simulink model "t_drone"  (R2025b)
settings: Solver=ode23t  StartTime=0.0  StopTime=timespot_spl(end)+2  FixedStep=0.01  MaxStep=1e-2  MinStep=1e-13  RelTol=1e-3  AbsTol=1e-3
InitFcn:
  | model = gcs;
  | 
  | configs = evalin('base', get_param([model '/Configurations'], 'Value'));
  | hold_time = evalin('base', get_param([model '/Hold Time'], 'Value'));
  | transistion_time = evalin('base', get_param([model '/Transistion Time'], 'Value'));
  | 
  | if exist('transforms', 'var') == 1
  |     transforms = transforms;
  | else
  |     transforms = false;
  | end
  | 
  | set_drone_configurations
model workspace (MATLAB code in the model file):
  | load('xy_data_membrane.mat');
undefined symbols (not defined in the file): air_rho, battery, drone_leg, filtD_altitude, filtD_attitude, filtD_motor, filtD_pitch, filtD_position, filtD_roll, filtD_yaw, filtM_altitude, filtM_attitude, filtM_pitch, filtM_position, filtM_roll, filtM_yaw, filtSpd_motor, kd_altitude, kd_attitude, kd_motor, kd_pitch, kd_position, kd_roll, kd_yaw, ki_altitude, ki_attitude, ki_motor, ki_pitch, ki_position, ki_roll, ki_yaw, kp_altitude, kp_attitude, kp_motor, kp_pitch, kp_position, kp_roll, kp_yaw, limit_altitude, limit_attitude, limit_motor, limit_pitch, limit_roll, limit_yaw, mass, pkgDensity, pkgSize, planedepth, pos2attitude, propeller, qc_motor, qd_area, qd_drag, spline_data, spline_yaw, timespot_spl, timespots, waypoints, wind_speed, X ... (+2)
libraries: sm_lib x176, nesl_utility x46, fl_lib x37, slpidlib x9, ee_lib x5, simulink_extras x4, sdl_lib x4, simulink x2, batteryecm_lib x1
(part 4 of 8)

== system t_drone/Quadcopter/Ground ==
  Ground : Subsystem  mask{waypoints=waypoints}
      mask prompts: waypoints "Waypoints [xyz] (m)"
      mask init:
      | plane_x = max(waypoints(1,:))-min(waypoints(1,:))+6;
      | plane_y = max(waypoints(2,:))-min(waypoints(2,:))+6;
      | 
      | offset_x = plane_x/2+min(waypoints(1,:))-3;
      | offset_y = plane_y/2+min(waypoints(2,:))-3;
  Infinite Plane : sm_lib/Curves and Surfaces/Infinite Plane  GraphicType=None  GraphicPlaneWidth=1  GraphicPlaneWidthUnits=m  GraphicPlaneHeight=1  GraphicPlaneHeightUnits=m  GraphicVisPropType=SimpleVisualProperties  GraphicDiffuseColor=[0.5 0.5 0.5]  GraphicOpacity=0  GraphicSpecularColor=[0.5 0.5 0.5 1.0]  GraphicAmbientColor=[0.15 0.15 0.15 1.0]  GraphicEmissiveColor=[0.0 0.0 0.0 1.0]  GraphicShininess=75
  Launch Insignia : sm_lib/Body Elements/Extruded Solid  ExtrusionType=General  PolygonNumSides=3  PolygonOuterRadius=1  PolygonOuterRadiusUnits=m  ExportEntireGeometry=off  ExtrusionCrossSection=[0.15 0.15; -0.15 0.15; -0.15 0.75; -0.6 0.75; -0.6 -0.75; -0.15 -0.75; -0.15 -0.15; 0.15 -0.15; 0.15 -0.75; 0.6 -0.75; 0.6 0.75; 0.15 0.75]*0.5  ExtrusionCrossSectionUnits=m  ExportConvexHullGeometry=off  ExtrusionLength=0.002  ExtrusionLengthUnits=m  InertiaType=CalculateFromGeometry  BasedOnType=Density  Density=1  DensityUnits=kg/m^3  Mass=1  MassUnits=kg  CenterOfMass=[0 0 0]  CenterOfMassUnits=m  MomentsOfInertia=[1 1 1]  MomentsOfInertiaUnits=kg*m^2  ProductsOfInertia=[0 0 0]  ProductsOfInertiaUnits=kg*m^2  GraphicType=FromGeometry  MarkerShape=Sphere  MarkerSize=10  GraphicVisPropType=SimpleVisualProperties  GraphicDiffuseColor=[0.3 0.3 0.3]  GraphicOpacity=1.0  GraphicSpecularColor=[0.5 0.5 0.5 1.0]  GraphicAmbientColor=[0.15 0.15 0.15 1.0]  GraphicEmissiveColor=[0.0 0.0 0.0 1.0]  GraphicShininess=75  DoExposeReferenceFrame=on  SerializedFrames=<Frames/>
  Launch Ring : sm_lib/Body Elements/Revolved Solid  RevolutionCrossSection=[0.5 0.001; 0.5 -0.001; 0.75 -0.001; 0.75 0.001]  RevolutionCrossSectionUnits=m  RevolutionExtent=Full  RevolutionAngle=180  RevolutionAngleUnits=deg  ExportConvexHullGeometry=off  InertiaType=CalculateFromGeometry  BasedOnType=Density  Density=1000  DensityUnits=kg/m^3  Mass=1  MassUnits=kg  CenterOfMass=[0 0 0]  CenterOfMassUnits=m  MomentsOfInertia=[1 1 1]  MomentsOfInertiaUnits=kg*m^2  ProductsOfInertia=[0 0 0]  ProductsOfInertiaUnits=kg*m^2  GraphicType=FromGeometry  MarkerShape=Sphere  MarkerSize=10  GraphicVisPropType=SimpleVisualProperties  GraphicDiffuseColor=[0.3 0.3 0.3]  GraphicOpacity=1.0  GraphicSpecularColor=[0.5 0.5 0.5 1.0]  GraphicAmbientColor=[0.15 0.15 0.15 1.0]  GraphicEmissiveColor=[0.0 0.0 0.0 1.0]  GraphicShininess=75  DoExposeReferenceFrame=on  SerializedFrames=<Frames/>
  Obstacles2 : Subsystem  VariantControl=show_obstacles
  Target Inner Ring : sm_lib/Body Elements/Revolved Solid  RevolutionCrossSection=[0.5 0.001; 0.5 -0.001; 0.75 -0.001; 0.75 0.001]*0.25  RevolutionCrossSectionUnits=m  RevolutionExtent=Full  RevolutionAngle=180  RevolutionAngleUnits=deg  ExportConvexHullGeometry=off  InertiaType=CalculateFromGeometry  BasedOnType=Density  Density=1000  DensityUnits=kg/m^3  Mass=1  MassUnits=kg  CenterOfMass=[0 0 0]  CenterOfMassUnits=m  MomentsOfInertia=[1 1 1]  MomentsOfInertiaUnits=kg*m^2  ProductsOfInertia=[0 0 0]  ProductsOfInertiaUnits=kg*m^2  GraphicType=FromGeometry  MarkerShape=Sphere  MarkerSize=10  GraphicVisPropType=SimpleVisualProperties  GraphicDiffuseColor=[1.0 0.2 0.2]  GraphicOpacity=1.0  GraphicSpecularColor=[0.5 0.5 0.5 1.0]  GraphicAmbientColor=[0.15 0.15 0.15 1.0]  GraphicEmissiveColor=[0.0 0.0 0.0 1.0]  GraphicShininess=75  DoExposeReferenceFrame=on  SerializedFrames=<Frames/>
  Target Middle Ring : sm_lib/Body Elements/Revolved Solid  RevolutionCrossSection=[0.5 0.001; 0.5 -0.001; 0.75 -0.001; 0.75 0.001]*0.5  RevolutionCrossSectionUnits=m  RevolutionExtent=Full  RevolutionAngle=180  RevolutionAngleUnits=deg  ExportConvexHullGeometry=off  InertiaType=CalculateFromGeometry  BasedOnType=Density  Density=1000  DensityUnits=kg/m^3  Mass=1  MassUnits=kg  CenterOfMass=[0 0 0]  CenterOfMassUnits=m  MomentsOfInertia=[1 1 1]  MomentsOfInertiaUnits=kg*m^2  ProductsOfInertia=[0 0 0]  ProductsOfInertiaUnits=kg*m^2  GraphicType=FromGeometry  MarkerShape=Sphere  MarkerSize=10  GraphicVisPropType=SimpleVisualProperties  GraphicDiffuseColor=[1.0 0.8 0.2]  GraphicOpacity=1.0  GraphicSpecularColor=[0.5 0.5 0.5 1.0]  GraphicAmbientColor=[0.15 0.15 0.15 1.0]  GraphicEmissiveColor=[0.0 0.0 0.0 1.0]  GraphicShininess=75  DoExposeReferenceFrame=on  SerializedFrames=<Frames/>
  Target Outer Ring : sm_lib/Body Elements/Revolved Solid  RevolutionCrossSection=[0.5 0.001; 0.5 -0.001; 0.75 -0.001; 0.75 0.001]  RevolutionCrossSectionUnits=m  RevolutionExtent=Full  RevolutionAngle=180  RevolutionAngleUnits=deg  ExportConvexHullGeometry=off  InertiaType=CalculateFromGeometry  BasedOnType=Density  Density=1000  DensityUnits=kg/m^3  Mass=1  MassUnits=kg  CenterOfMass=[0 0 0]  CenterOfMassUnits=m  MomentsOfInertia=[1 1 1]  MomentsOfInertiaUnits=kg*m^2  ProductsOfInertia=[0 0 0]  ProductsOfInertiaUnits=kg*m^2  GraphicType=FromGeometry  MarkerShape=Sphere  MarkerSize=10  GraphicVisPropType=SimpleVisualProperties  GraphicDiffuseColor=[0.2 0.4 1.0]  GraphicOpacity=1.0  GraphicSpecularColor=[0.5 0.5 0.5 1.0]  GraphicAmbientColor=[0.15 0.15 0.15 1.0]  GraphicEmissiveColor=[0.0 0.0 0.0 1.0]  GraphicShininess=75  DoExposeReferenceFrame=on  SerializedFrames=<Frames/>
  Trajectory : Subsystem
  Transform Launch : sm_lib/Frames and Transforms/Rigid Transform  RotationMethod=None  FollAlignAxisA=+X  BaseAlignAxisA=+Y  FollAlignAxisB=+Y  BaseAlignAxisB=+Z  RotationStandardAxis=+Z  RotationAngle=0.0  RotationAngleUnits=deg  RotationArbitraryAxis=[0 0 1]  RotationSequenceAxes=FollowerAxes  RotationSequence=XYX  RotationSequenceAngles=[0 0 0]  RotationSequenceAnglesUnits=deg  RotationMatrix=[1 0 0; 0 1 0; 0 0 1]  Quaternion=[1 0 0 0]  TranslationMethod=Cartesian  TranslationCartesianOffset=[waypoints(1:2,1)' 0 ]  TranslationCartesianOffsetUnits=m  TranslationStandardAxis=+Z  TranslationStandardOffset=0  TranslationStandardOffsetUnits=m  TranslationROffset=0  TranslationROffsetUnits=m  TranslationThetaOffset=0  TranslationThetaOffsetUnits=deg  TranslationZOffset=0  TranslationZOffsetUnits=m
  Transform Target : sm_lib/Frames and Transforms/Rigid Transform  RotationMethod=None  FollAlignAxisA=+X  BaseAlignAxisA=+Y  FollAlignAxisB=+Y  BaseAlignAxisB=+Z  RotationStandardAxis=+Z  RotationAngle=0.0  RotationAngleUnits=deg  RotationArbitraryAxis=[0 0 1]  RotationSequenceAxes=FollowerAxes  RotationSequence=XYX  RotationSequenceAngles=[0 0 0]  RotationSequenceAnglesUnits=deg  RotationMatrix=[1 0 0; 0 1 0; 0 0 1]  Quaternion=[1 0 0 0]  TranslationMethod=Cartesian  TranslationCartesianOffset=[waypoints(1:2,end)' 0 ]  TranslationCartesianOffsetUnits=m  TranslationStandardAxis=+Z  TranslationStandardOffset=0  TranslationStandardOffsetUnits=m  TranslationROffset=0  TranslationROffsetUnits=m  TranslationThetaOffset=0  TranslationThetaOffsetUnits=deg  TranslationZOffset=0  TranslationZOffsetUnits=m
  Variant Connector : VariantPMConnector  VariantControls=__PRM__SERIALIZED__DATA__:show_obstacles == true
  W : PMIOPort  Side=Right
  G : PMIOPort  Port=2  Side=Left
  connections:
  W/RConn1 -- Ground/LConn1 -- Transform Launch/LConn1 -- Transform Target/LConn1 -- Trajectory/RConn1
  Target Middle Ring/RConn1 -- Target Inner Ring/RConn1 -- Transform Target/RConn1 -- Target Outer Ring/RConn1
  Infinite Plane/LConn1 -- Ground/RConn1
  Infinite Plane/RConn1 -- G/RConn1
  Launch Ring/RConn1 -- Variant Connector/RConn1 -- Transform Launch/RConn1 -- Launch Insignia/RConn1
  Variant Connector/LConn1 -- Obstacles2/LConn1

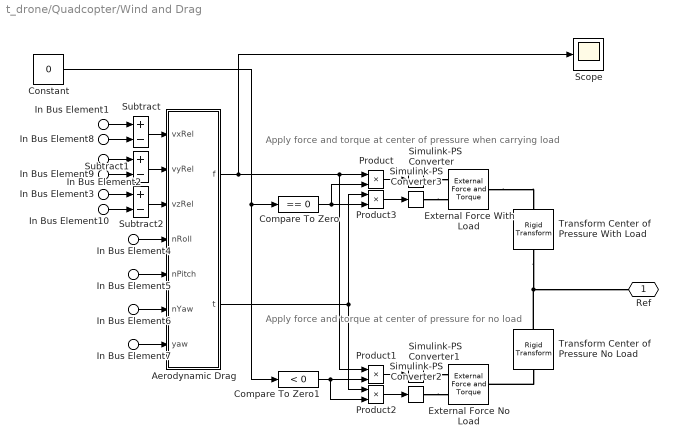
== system t_drone/Quadcopter/Wind and Drag ==
  note: Apply force and torque at center of pressure when carrying load
  note: Apply force and torque at center of pressure for no load
  In Bus Element8 : Inport  PortName=Env  Element=vx
  In Bus Element9 : Inport  PortName=Env  Element=vy
  In Bus Element10 : Inport  PortName=Env  Element=vz
  In Bus Element1 : Inport  Port=2  PortName=Cha  Element=vx
  In Bus Element2 : Inport  Port=2  PortName=Cha  Element=vy
  In Bus Element3 : Inport  Port=2  PortName=Cha  Element=vz
  In Bus Element4 : Inport  Port=2  PortName=Cha  Element=nRoll
  In Bus Element5 : Inport  Port=2  PortName=Cha  Element=nPitch
  In Bus Element6 : Inport  Port=2  PortName=Cha  Element=nYaw
  In Bus Element7 : Inport  Port=2  PortName=Cha  Element=yaw
  Aerodynamic Drag : Subsystem  mask{drag_coeff=qd_drag, area_values=qd_area, rho_air=air_rho}
      mask prompts: drag_coeff "Drag Coefficients"; area_values "Area Values (m^2)"; rho_air "Air Density"
  Compare To Zero : simulink/Logic and Bit Operations/Compare To Zero  relop===  OutDataTypeStr=uint8  ZeroCross=off
  Compare To Zero1 : simulink/Logic and Bit Operations/Compare To Zero  relop=<  OutDataTypeStr=uint8  ZeroCross=off
  Constant : Constant  Value=0
  External Force No Load : sm_lib/Forces and Torques/External Force and Torque  EnableForceX=off  EnableForceY=off  EnableForceZ=off  EnableForce=on  ForceResolutionFrame=World  EnableTorqueX=off  EnableTorqueY=off  EnableTorqueZ=off  EnableTorque=on  TorqueResolutionFrame=AttachedFrame
  External Force With Load : sm_lib/Forces and Torques/External Force and Torque  EnableForceX=off  EnableForceY=off  EnableForceZ=off  EnableForce=on  ForceResolutionFrame=World  EnableTorqueX=off  EnableTorqueY=off  EnableTorqueZ=off  EnableTorque=on  TorqueResolutionFrame=AttachedFrame
  Product{,1..3} (4 alike) : Product
  Scope : Scope
      settings: ActiveDisplayYMinimum=-0.40984  ActiveDisplayYMaximum=3.52459
  Simulink-PS Converter{,1..3} (4 alike) : nesl_utility/Simulink-PS Converter  PhysicalDomain=network_engine_domain  SubClassName=ps_input  LeftPortType=input  RightPortType=output  PseudoPeriodic=off  Frequencies=[]  NoiseDistribution=none  NoiseParameters=[]  Unit=1  AffineConversion=off  FilteringAndDerivatives=provide  SimscapeFilterOrder=1  InputFilterTimeConstant=0.001  UdotUserProvided=0
  Subtract : Sum  Inputs=+-
  Subtract1 : Sum  Inputs=+-
  Subtract2 : Sum  Inputs=+-
  Transform Center of Pressure No Load : sm_lib/Frames and Transforms/Rigid Transform  RotationMethod=None  FollAlignAxisA=+X  BaseAlignAxisA=+Y  FollAlignAxisB=+Y  BaseAlignAxisB=+Z  RotationStandardAxis=+Z  RotationAngle=0.0  RotationAngleUnits=deg  RotationArbitraryAxis=[0 0 1]  RotationSequenceAxes=FollowerAxes  RotationSequence=XYX  RotationSequenceAngles=[0 0 0]  RotationSequenceAnglesUnits=deg  RotationMatrix=[1 0 0; 0 1 0; 0 0 1]  Quaternion=[1 0 0 0]  TranslationMethod=None  TranslationCartesianOffset=[0 0 0]  TranslationCartesianOffsetUnits=m  TranslationStandardAxis=+Z  TranslationStandardOffset=0  TranslationStandardOffsetUnits=m  TranslationROffset=0  TranslationROffsetUnits=m  TranslationThetaOffset=0  TranslationThetaOffsetUnits=deg  TranslationZOffset=0  TranslationZOffsetUnits=m
  Transform Center of Pressure With Load : sm_lib/Frames and Transforms/Rigid Transform  RotationMethod=None  FollAlignAxisA=+X  BaseAlignAxisA=+Y  FollAlignAxisB=+Y  BaseAlignAxisB=+Z  RotationStandardAxis=+Z  RotationAngle=0.0  RotationAngleUnits=deg  RotationArbitraryAxis=[0 0 1]  RotationSequenceAxes=FollowerAxes  RotationSequence=XYX  RotationSequenceAngles=[0 0 0]  RotationSequenceAnglesUnits=deg  RotationMatrix=[1 0 0; 0 1 0; 0 0 1]  Quaternion=[1 0 0 0]  TranslationMethod=StandardAxis  TranslationCartesianOffset=[0 0 0]  TranslationCartesianOffsetUnits=m  TranslationStandardAxis=+Z  TranslationStandardOffset=-pkgSize(3)/2  TranslationStandardOffsetUnits=m  TranslationROffset=0  TranslationROffsetUnits=m  TranslationThetaOffset=0  TranslationThetaOffsetUnits=deg  TranslationZOffset=0  TranslationZOffsetUnits=m
  Ref : PMIOPort  Side=Right
  wires:
  Product/1 -> Simulink-PS Converter/1
  Product1/1 -> Simulink-PS Converter1/1
  Constant/1 -> Compare To Zero1/1, Compare To Zero/1
  Compare To Zero/1 -> Product/2, Product3/2
  Compare To Zero1/1 -> Product2/2, Product1/2
  In Bus Element1/1 -> Subtract/1
  In Bus Element8/1 -> Subtract/2
  In Bus Element7/1 -> Aerodynamic Drag/7(yaw)
  In Bus Element2/1 -> Subtract1/1
  In Bus Element9/1 -> Subtract1/2
  Subtract/1 -> Aerodynamic Drag/1(vxRel)
  Subtract1/1 -> Aerodynamic Drag/2(vyRel)
  In Bus Element3/1 -> Subtract2/1
  In Bus Element10/1 -> Subtract2/2
  Subtract2/1 -> Aerodynamic Drag/3(vzRel)
  In Bus Element4/1 -> Aerodynamic Drag/4(nRoll)
  In Bus Element5/1 -> Aerodynamic Drag/5(nPitch)
  In Bus Element6/1 -> Aerodynamic Drag/6(nYaw)
  Product2/1 -> Simulink-PS Converter2/1
  Product3/1 -> Simulink-PS Converter3/1
  Aerodynamic Drag/1(f) -> Scope/1, Product1/1, Product/1
  Aerodynamic Drag/2(t) -> Product3/1, Product2/1
  connections:
  Transform Center of Pressure With Load/LConn1 -- Transform Center of Pressure No Load/LConn1 -- Ref/RConn1
  Transform Center of Pressure No Load/RConn1 -- External Force No Load/RConn1
  External Force With Load/RConn1 -- Transform Center of Pressure With Load/RConn1
  Simulink-PS Converter/RConn1 -- External Force With Load/LConn1
  Simulink-PS Converter1/RConn1 -- External Force No Load/LConn1
  Simulink-PS Converter2/RConn1 -- External Force No Load/LConn2
  Simulink-PS Converter3/RConn1 -- External Force With Load/LConn2

== system t_drone/Reference/Derivative ==
  des xyz : Inport
  Demux : Demux  Outputs=3
  Derivative : Derivative
  Derivative1 : Derivative
  Derivative2 : Derivative
  Mux1 : Mux  Inputs=3
  des_vel : Outport
  wires:
  Demux/1 -> Derivative/1
  Mux1/1 -> des_vel/1  "des_vel"
  des xyz/1 -> Demux/1
  Demux/2 -> Derivative1/1
  Demux/3 -> Derivative2/1
  Derivative2/1 -> Mux1/3
  Derivative/1 -> Mux1/1
  Derivative1/1 -> Mux1/2

== system t_drone/Reference/Interpolate Spline Points ==
  In1 : Inport
  Constant : Constant  Value=timespot_spl(end)
  Lookup Linear Interpolation1 : Lookup_n-D  NumberOfTableDimensions=1  BreakpointsForDimension1=timespot_spl  Table=spline_yaw  InterpMethod=Akima spline  ExtrapMethod=Clip  InternalRulePriority=Speed  RndMeth=Simplest
  Lookup Linear Interpolation4 : Lookup_n-D  NumberOfTableDimensions=1  BreakpointsForDimension1=timespot_spl  Table=spline_data(:,1)  InterpMethod=Cubic spline  ExtrapMethod=Clip  InternalRulePriority=Speed  RndMeth=Simplest
  Lookup Linear Interpolation5 : Lookup_n-D  NumberOfTableDimensions=1  BreakpointsForDimension1=timespot_spl  Table=spline_data(:,2)  InterpMethod=Cubic spline  ExtrapMethod=Clip  InternalRulePriority=Speed  RndMeth=Simplest
  Lookup Linear Interpolation6 : Lookup_n-D  NumberOfTableDimensions=1  BreakpointsForDimension1=timespot_spl  Table=spline_data(:,3)  InterpMethod=Cubic spline  ExtrapMethod=Clip  InternalRulePriority=Speed  RndMeth=Simplest
  Min : MinMax  Inputs=2
  Mux2 : Mux  Inputs=3
  Yaw : Outport
  des_pos : Outport  Port=2
  wires:
  Mux2/1 -> des_pos/1  "des_pos"
  Min/1 -> Lookup Linear Interpolation6/1, Lookup Linear Interpolation5/1, Lookup Linear Interpolation1/1, Lookup Linear Interpolation4/1
  Lookup Linear Interpolation5/1 -> Mux2/2
  Lookup Linear Interpolation4/1 -> Mux2/1
  Lookup Linear Interpolation6/1 -> Mux2/3
  Lookup Linear Interpolation1/1 -> Yaw/1
  In1/1 -> Min/1
  Constant/1 -> Min/2

== system t_drone/Maneuver Controller/Altitude and YPR Control/Control Pitch ==
  PID Input : Inport
  From Workspace : FromWorkspace  VariableName=ts_p  OutputAfterFinalValue=Holding final value
  From Workspace1 : FromWorkspace  VariableName=ts_i  OutputAfterFinalValue=Holding final value
  From Workspace2 : FromWorkspace  VariableName=ts_d  OutputAfterFinalValue=Holding final value
  From Workspace3 : FromWorkspace  VariableName=ts_f  OutputAfterFinalValue=Holding final value
  From Workspace4 : FromWorkspace  VariableName=ts_l  OutputAfterFinalValue=Holding final value
  Gain : Gain  Gain=-1
  PID Controller : slpidlib/PID Controller  Controller=PID  Form=Parallel  TimeDomain=Continuous-time  UseExternalTs=off  SampleTime=-1  IntegratorMethod=Forward Euler  FilterMethod=Forward Euler  ControllerParametersSource=external  P=1  I=1  UseKiTs=off  D=0  UseExternalDerivativeSource=off  N=100  UseFilter=on  TunerSelectOption=Transfer Function Based (PID Tuner App)  InitialConditionSource=internal  InitialConditionForIntegrator=0  InitialConditionForFilter=0  DifferentiatorICPrevScaledInput=0  ExternalReset=none  TrackingMode=off  Kt=1  LimitOutput=on  SatLimitsSource=external  UpperSaturationLimit=inf  LowerSaturationLimit=-inf  LinearizeAsGain=on  AntiWindupMode=none  Kb=1  LimitIntegrator=off  UpperIntegratorSaturationLimit=inf  LowerIntegratorSaturationLimit=-inf  POutMin=[]  POutMax=[]  IOutMin=[]  IOutMax=[]  DOutMin=[]  DOutMax=[]  NOutMin=[]  NOutMax=[]  SumOutMin=[]  SumOutMax=[]  SaturationOutMin=[]  SaturationOutMax=[]  PParamMin=[]  PParamMax=[]  IParamMin=[]  IParamMax=[]  DParamMin=[]  DParamMax=[]  NParamMin=[]  NParamMax=[]  KbParamMin=[]  KbParamMax=[]  KtParamMin=[]  KtParamMax=[]  KbOutMin=[]  KbOutMax=[]  KtOutMin=[]  KtOutMax=[]  IntegratorOutMin=[]  IntegratorOutMax=[]  FilterOutMin=[]  FilterOutMax=[]  SumI1OutMin=[]  SumI1OutMax=[]  SumI2OutMin=[]  SumI2OutMax=[]  SumI3OutMin=[]  SumI3OutMax=[]  SumI4OutMin=[]  SumI4OutMax=[]  SumDOutMin=[]  SumDOutMax=[]  DifferentiatorOutMin=[]  DifferentiatorOutMax=[]  FilterDiffOutCoefMin=[]  FilterDiffOutCoefMax=[]  ReciprocalOutMin=[]  ReciprocalOutMax=[]  SumDenOutMin=[]  SumDenOutMax=[]  SumNumOutMin=[]  SumNumOutMax=[]  DivideOutMin=[]  DivideOutMax=[]  UdiffTsProdOutMin=[]  UdiffTsProdOutMax=[]  NTsProdOutMin=[]  NTsProdOutMax=[]  UintegralTsProdOutMin=[]  UintegralTsProdOutMax=[]  UngainTsProdOutMin=[]  UngainTsProdOutMax=[]  ClampingZeroOutDataTypeStr=Inherit: Inherit via back propagation  ClampingZeroOutMin=[]  ClampingZeroOutMax=[]  FilterDenConstantOutDataTypeStr=Inherit: Inherit via back propagation  FilterDenConstantOutMin=[]  FilterDenConstantOutMax=[]  PCopyOutDataTypeStr=Inherit: Inherit via back propagation  PCopyOutMin=[]  PCopyOutMax=[]  NCopyOutDataTypeStr=Inherit: Inherit via back propagation  NCopyOutMin=[]  NCopyOutMax=[]  IntegratorContinuousStateAttributes=''  IntegratorStateMustResolveToSignalObject=off  IntegratorRTWStateStorageClass=Auto  FilterContinuousStateAttributes=''  FilterStateMustResolveToSignalObject=off  FilterRTWStateStorageClass=Auto  ParallelPVariant=ExternalParameters  IdealPVariant=Disabled  IVariant=ExternalParameters  DVariant=ExternalParameters  IntegratorVariant=Continuous  SatVariant=External  AWVariant=Passthrough  PCopyVariant=Disabled  TRVariant=Disabled  FdbkBlocksVariant=Forward  IdealPFdbkVariant=Disabled  SatFdbkVariant=Disabled  DerivativeFilterVariant=ContFilter  NVariant=ExternalParameters  NCopyVariant=Disabled  FilterICVariant=InternalICsFilter  IntegratorICVariant=InternalICs  ExternalResetVariant=Disabled  TRSumVariant=Passthrough  SumFdbkVariant=Disabled  SumVariant=Sum_PID  TsampFilterVariant=InternalTs  TsampNgainVariant=Passthrough  TsampIntegralVariant=Disabled_SignalSpec  ExternalSaturationOutDataTypeStr=Inherit: Same as second input  DerivativeSourceVariant=ErrorSignal  PreIntVariant=InternalPreInt
  PID Out : Outport
  wires:
  PID Input/1 -> PID Controller/1
  PID Controller/1 -> PID Out/1
  From Workspace/1 -> PID Controller/2
  From Workspace1/1 -> PID Controller/3
  From Workspace2/1 -> PID Controller/4
  From Workspace3/1 -> PID Controller/5
  From Workspace4/1 -> Gain/1, PID Controller/6
  Gain/1 -> PID Controller/7

== system t_drone/Maneuver Controller/Altitude and YPR Control/Control Roll ==
  PID Input : Inport
  From Workspace : FromWorkspace  VariableName=ts_p  OutputAfterFinalValue=Holding final value
  From Workspace1 : FromWorkspace  VariableName=ts_i  OutputAfterFinalValue=Holding final value
  From Workspace2 : FromWorkspace  VariableName=ts_d  OutputAfterFinalValue=Holding final value
  From Workspace3 : FromWorkspace  VariableName=ts_f  OutputAfterFinalValue=Holding final value
  From Workspace4 : FromWorkspace  VariableName=ts_l  OutputAfterFinalValue=Holding final value
  Gain : Gain  Gain=-1
  PID Controller : slpidlib/PID Controller  Controller=PID  Form=Parallel  TimeDomain=Continuous-time  UseExternalTs=off  SampleTime=-1  IntegratorMethod=Forward Euler  FilterMethod=Forward Euler  ControllerParametersSource=external  P=1  I=1  UseKiTs=off  D=0  UseExternalDerivativeSource=off  N=100  UseFilter=on  TunerSelectOption=Transfer Function Based (PID Tuner App)  InitialConditionSource=internal  InitialConditionForIntegrator=0  InitialConditionForFilter=0  DifferentiatorICPrevScaledInput=0  ExternalReset=none  TrackingMode=off  Kt=1  LimitOutput=on  SatLimitsSource=external  UpperSaturationLimit=inf  LowerSaturationLimit=-inf  LinearizeAsGain=on  AntiWindupMode=none  Kb=1  LimitIntegrator=off  UpperIntegratorSaturationLimit=inf  LowerIntegratorSaturationLimit=-inf  POutMin=[]  POutMax=[]  IOutMin=[]  IOutMax=[]  DOutMin=[]  DOutMax=[]  NOutMin=[]  NOutMax=[]  SumOutMin=[]  SumOutMax=[]  SaturationOutMin=[]  SaturationOutMax=[]  PParamMin=[]  PParamMax=[]  IParamMin=[]  IParamMax=[]  DParamMin=[]  DParamMax=[]  NParamMin=[]  NParamMax=[]  KbParamMin=[]  KbParamMax=[]  KtParamMin=[]  KtParamMax=[]  KbOutMin=[]  KbOutMax=[]  KtOutMin=[]  KtOutMax=[]  IntegratorOutMin=[]  IntegratorOutMax=[]  FilterOutMin=[]  FilterOutMax=[]  SumI1OutMin=[]  SumI1OutMax=[]  SumI2OutMin=[]  SumI2OutMax=[]  SumI3OutMin=[]  SumI3OutMax=[]  SumI4OutMin=[]  SumI4OutMax=[]  SumDOutMin=[]  SumDOutMax=[]  DifferentiatorOutMin=[]  DifferentiatorOutMax=[]  FilterDiffOutCoefMin=[]  FilterDiffOutCoefMax=[]  ReciprocalOutMin=[]  ReciprocalOutMax=[]  SumDenOutMin=[]  SumDenOutMax=[]  SumNumOutMin=[]  SumNumOutMax=[]  DivideOutMin=[]  DivideOutMax=[]  UdiffTsProdOutMin=[]  UdiffTsProdOutMax=[]  NTsProdOutMin=[]  NTsProdOutMax=[]  UintegralTsProdOutMin=[]  UintegralTsProdOutMax=[]  UngainTsProdOutMin=[]  UngainTsProdOutMax=[]  ClampingZeroOutDataTypeStr=Inherit: Inherit via back propagation  ClampingZeroOutMin=[]  ClampingZeroOutMax=[]  FilterDenConstantOutDataTypeStr=Inherit: Inherit via back propagation  FilterDenConstantOutMin=[]  FilterDenConstantOutMax=[]  PCopyOutDataTypeStr=Inherit: Inherit via back propagation  PCopyOutMin=[]  PCopyOutMax=[]  NCopyOutDataTypeStr=Inherit: Inherit via back propagation  NCopyOutMin=[]  NCopyOutMax=[]  IntegratorContinuousStateAttributes=''  IntegratorStateMustResolveToSignalObject=off  IntegratorRTWStateStorageClass=Auto  FilterContinuousStateAttributes=''  FilterStateMustResolveToSignalObject=off  FilterRTWStateStorageClass=Auto  ParallelPVariant=ExternalParameters  IdealPVariant=Disabled  IVariant=ExternalParameters  DVariant=ExternalParameters  IntegratorVariant=Continuous  SatVariant=External  AWVariant=Passthrough  PCopyVariant=Disabled  TRVariant=Disabled  FdbkBlocksVariant=Forward  IdealPFdbkVariant=Disabled  SatFdbkVariant=Disabled  DerivativeFilterVariant=ContFilter  NVariant=ExternalParameters  NCopyVariant=Disabled  FilterICVariant=InternalICsFilter  IntegratorICVariant=InternalICs  ExternalResetVariant=Disabled  TRSumVariant=Passthrough  SumFdbkVariant=Disabled  SumVariant=Sum_PID  TsampFilterVariant=InternalTs  TsampNgainVariant=Passthrough  TsampIntegralVariant=Disabled_SignalSpec  ExternalSaturationOutDataTypeStr=Inherit: Same as second input  DerivativeSourceVariant=ErrorSignal  PreIntVariant=InternalPreInt
  PID Out : Outport
  wires:
  PID Input/1 -> PID Controller/1
  PID Controller/1 -> PID Out/1
  From Workspace/1 -> PID Controller/2
  From Workspace1/1 -> PID Controller/3
  From Workspace2/1 -> PID Controller/4
  From Workspace3/1 -> PID Controller/5
  From Workspace4/1 -> Gain/1, PID Controller/6
  Gain/1 -> PID Controller/7

== system t_drone/Maneuver Controller/Altitude and YPR Control/Control Yaw ==
  PID Input : Inport
  From Workspace : FromWorkspace  VariableName=ts_p  OutputAfterFinalValue=Holding final value
  From Workspace1 : FromWorkspace  VariableName=ts_i  OutputAfterFinalValue=Holding final value
  From Workspace2 : FromWorkspace  VariableName=ts_d  OutputAfterFinalValue=Holding final value
  From Workspace3 : FromWorkspace  VariableName=ts_f  OutputAfterFinalValue=Holding final value
  From Workspace4 : FromWorkspace  VariableName=ts_l  OutputAfterFinalValue=Holding final value
  Gain : Gain  Gain=-1
  PID Controller : slpidlib/PID Controller  Controller=PID  Form=Parallel  TimeDomain=Continuous-time  UseExternalTs=off  SampleTime=-1  IntegratorMethod=Forward Euler  FilterMethod=Forward Euler  ControllerParametersSource=external  P=1  I=1  UseKiTs=off  D=0  UseExternalDerivativeSource=off  N=100  UseFilter=on  TunerSelectOption=Transfer Function Based (PID Tuner App)  InitialConditionSource=internal  InitialConditionForIntegrator=0  InitialConditionForFilter=0  DifferentiatorICPrevScaledInput=0  ExternalReset=none  TrackingMode=off  Kt=1  LimitOutput=on  SatLimitsSource=external  UpperSaturationLimit=inf  LowerSaturationLimit=-inf  LinearizeAsGain=on  AntiWindupMode=none  Kb=1  LimitIntegrator=off  UpperIntegratorSaturationLimit=inf  LowerIntegratorSaturationLimit=-inf  POutMin=[]  POutMax=[]  IOutMin=[]  IOutMax=[]  DOutMin=[]  DOutMax=[]  NOutMin=[]  NOutMax=[]  SumOutMin=[]  SumOutMax=[]  SaturationOutMin=[]  SaturationOutMax=[]  PParamMin=[]  PParamMax=[]  IParamMin=[]  IParamMax=[]  DParamMin=[]  DParamMax=[]  NParamMin=[]  NParamMax=[]  KbParamMin=[]  KbParamMax=[]  KtParamMin=[]  KtParamMax=[]  KbOutMin=[]  KbOutMax=[]  KtOutMin=[]  KtOutMax=[]  IntegratorOutMin=[]  IntegratorOutMax=[]  FilterOutMin=[]  FilterOutMax=[]  SumI1OutMin=[]  SumI1OutMax=[]  SumI2OutMin=[]  SumI2OutMax=[]  SumI3OutMin=[]  SumI3OutMax=[]  SumI4OutMin=[]  SumI4OutMax=[]  SumDOutMin=[]  SumDOutMax=[]  DifferentiatorOutMin=[]  DifferentiatorOutMax=[]  FilterDiffOutCoefMin=[]  FilterDiffOutCoefMax=[]  ReciprocalOutMin=[]  ReciprocalOutMax=[]  SumDenOutMin=[]  SumDenOutMax=[]  SumNumOutMin=[]  SumNumOutMax=[]  DivideOutMin=[]  DivideOutMax=[]  UdiffTsProdOutMin=[]  UdiffTsProdOutMax=[]  NTsProdOutMin=[]  NTsProdOutMax=[]  UintegralTsProdOutMin=[]  UintegralTsProdOutMax=[]  UngainTsProdOutMin=[]  UngainTsProdOutMax=[]  ClampingZeroOutDataTypeStr=Inherit: Inherit via back propagation  ClampingZeroOutMin=[]  ClampingZeroOutMax=[]  FilterDenConstantOutDataTypeStr=Inherit: Inherit via back propagation  FilterDenConstantOutMin=[]  FilterDenConstantOutMax=[]  PCopyOutDataTypeStr=Inherit: Inherit via back propagation  PCopyOutMin=[]  PCopyOutMax=[]  NCopyOutDataTypeStr=Inherit: Inherit via back propagation  NCopyOutMin=[]  NCopyOutMax=[]  IntegratorContinuousStateAttributes=''  IntegratorStateMustResolveToSignalObject=off  IntegratorRTWStateStorageClass=Auto  FilterContinuousStateAttributes=''  FilterStateMustResolveToSignalObject=off  FilterRTWStateStorageClass=Auto  ParallelPVariant=ExternalParameters  IdealPVariant=Disabled  IVariant=ExternalParameters  DVariant=ExternalParameters  IntegratorVariant=Continuous  SatVariant=External  AWVariant=Passthrough  PCopyVariant=Disabled  TRVariant=Disabled  FdbkBlocksVariant=Forward  IdealPFdbkVariant=Disabled  SatFdbkVariant=Disabled  DerivativeFilterVariant=ContFilter  NVariant=ExternalParameters  NCopyVariant=Disabled  FilterICVariant=InternalICsFilter  IntegratorICVariant=InternalICs  ExternalResetVariant=Disabled  TRSumVariant=Passthrough  SumFdbkVariant=Disabled  SumVariant=Sum_PID  TsampFilterVariant=InternalTs  TsampNgainVariant=Passthrough  TsampIntegralVariant=Disabled_SignalSpec  ExternalSaturationOutDataTypeStr=Inherit: Same as second input  DerivativeSourceVariant=ErrorSignal  PreIntVariant=InternalPreInt
  PID Out : Outport
  wires:
  PID Input/1 -> PID Controller/1
  PID Controller/1 -> PID Out/1
  From Workspace/1 -> PID Controller/2
  From Workspace1/1 -> PID Controller/3
  From Workspace2/1 -> PID Controller/4
  From Workspace3/1 -> PID Controller/5
  From Workspace4/1 -> Gain/1, PID Controller/6
  Gain/1 -> PID Controller/7

== system t_drone/Maneuver Controller/Altitude and YPR Control/Pause Motor ==
  note: Create pulse to briefly stop motor while package is dropped.
  y : Inport
  Bias : Bias  Bias=1  SaturateOnIntegerOverflow=off
  Delay : Delay  DelayLength=dur_pulse/ts_pulse  InitialCondition=0  SampleTime=ts_pulse
  Sign Change : Gain  Gain=-1
  Sum2 : Sum  Inputs=|+-  OutDataTypeStr=double  InputSameDT=on  SaturateOnIntegerOverflow=on
  En : Outport
  wires:
  Delay/1 -> Sum2/1
  Sum2/1 -> Bias/1
  y/1 -> Sign Change/1
  Sign Change/1 -> Delay/1, Sum2/2
  Bias/1 -> En/1

== system t_drone/Maneuver Controller/Altitude and YPR Control/Subsystem ==
  cmd : Inport
  load : Inport  Port=2
  Bias : Bias  Bias=+1  SaturateOnIntegerOverflow=off
  Bias Chassis : Bias  Bias=700  SaturateOnIntegerOverflow=off
  Bias Load : Gain  Gain=260*pkgSize(1)^3*pkgDensity
  Speed : Gain  Gain=2*pi
  Sum : Sum
  Out1 : Outport
  wires:
  cmd/1 -> Bias Chassis/1
  Speed/1 -> Out1/1
  load/1 -> Bias/1  "mode"
  Bias/1 -> Bias Load/1  "presence"
  Bias Load/1 -> Sum/2
  Bias Chassis/1 -> Sum/1
  Sum/1 -> Speed/1

== system t_drone/Maneuver Controller/Position Control/Filter ==
  i : Inport
  Demux1 : Demux  Outputs=3
  Mux p1 : Mux  Inputs=3
  Transfer Fcn : TransferFcn  Denominator=[filt_const 1]
  Transfer Fcn1 : TransferFcn  Denominator=[filt_const 1]
  Transfer Fcn2 : TransferFcn  Denominator=[filt_const 1]
  o : Outport
  wires:
  i/1 -> Demux1/1
  Transfer Fcn2/1 -> Mux p1/3
  Transfer Fcn1/1 -> Mux p1/2
  Demux1/3 -> Transfer Fcn2/1
  Transfer Fcn/1 -> Mux p1/1
  Demux1/2 -> Transfer Fcn1/1
  Demux1/1 -> Transfer Fcn/1
  Mux p1/1 -> o/1

== system t_drone/Quadcopter/6 DOF/Joints ==
  note: Separate joints used to permit definition of camera viewpoints that do not rotate with the quadcopter.
  Cartesian Joint : sm_lib/Joints/Cartesian Joint  JointMode=Normal  CompositeWrenchDir=FollowerOnBase  CompositeWrenchFrame=BaseFrame  SenseConstraintForce=off  SenseConstraintTorque=off  SenseTotalForce=off  SenseTotalTorque=off  PxPositionTargetSpecify=on  PxPositionTargetPriority=High  PxPositionTargetValue=waypoints(1,1)  PxPositionTargetValueUnits=m  PxVelocityTargetSpecify=off  PxVelocityTargetPriority=High  PxVelocityTargetValue=0  PxVelocityTargetValueUnits=m/s  PxEquilibriumPosition=0  PxEquilibriumPositionUnits=m  PxSpringStiffness=0  PxSpringStiffnessUnits=N/m  PxDampingCoefficient=0  PxDampingCoefficientUnits=N/(m/s)  PxLowerLimitSpecify=off  PxLowerLimitBound=-1  PxLowerLimitBoundUnits=m  PxLowerLimitStiffness=1e6  PxLowerLimitStiffnessUnits=N/m  PxLowerLimitDamping=1e3  PxLowerLimitDampingUnits=N/(m/s)  PxLowerLimitTransitionRegionWidth=1e-4  PxLowerLimitTransitionRegionWidthUnits=m  PxUpperLimitSpecify=off  PxUpperLimitBound=1  PxUpperLimitBoundUnits=m  PxUpperLimitStiffness=1e6  PxUpperLimitStiffnessUnits=N/m  PxUpperLimitDamping=1e3  PxUpperLimitDampingUnits=N/(m/s)  PxUpperLimitTransitionRegionWidth=1e-4  PxUpperLimitTransitionRegionWidthUnits=m  PxTorqueActuationMode=NoTorque  PxMotionActuationMode=ComputedMotion  PxSensePosition=on  PxSenseVelocity=on  PxSenseAcceleration=off  PxSenseTorqueForce=off  PxSenseLowerLimitTorqueForce=off  PxSenseUpperLimitTorqueForce=off  PyPositionTargetSpecify=on  PyPositionTargetPriority=High  PyPositionTargetValue=waypoints(2,1)  PyPositionTargetValueUnits=m  PyVelocityTargetSpecify=off  PyVelocityTargetPriority=High  PyVelocityTargetValue=0  PyVelocityTargetValueUnits=m/s  PyEquilibriumPosition=0  PyEquilibriumPositionUnits=m  PySpringStiffness=0  PySpringStiffnessUnits=N/m  PyDampingCoefficient=0  PyDampingCoefficientUnits=N/(m/s)  PyLowerLimitSpecify=off  PyLowerLimitBound=-1  PyLowerLimitBoundUnits=m  PyLowerLimitStiffness=1e6  PyLowerLimitStiffnessUnits=N/m  PyLowerLimitDamping=1e3  PyLowerLimitDampingUnits=N/(m/s)  PyLowerLimitTransitionRegionWidth=1e-4  PyLowerLimitTransitionRegionWidthUnits=m  PyUpperLimitSpecify=off  PyUpperLimitBound=1  PyUpperLimitBoundUnits=m  PyUpperLimitStiffness=1e6  PyUpperLimitStiffnessUnits=N/m  PyUpperLimitDamping=1e3  PyUpperLimitDampingUnits=N/(m/s)  PyUpperLimitTransitionRegionWidth=1e-4  PyUpperLimitTransitionRegionWidthUnits=m  PyTorqueActuationMode=NoTorque  PyMotionActuationMode=ComputedMotion  PySensePosition=on  PySenseVelocity=on  PySenseAcceleration=off  PySenseTorqueForce=off  PySenseLowerLimitTorqueForce=off  PySenseUpperLimitTorqueForce=off  PzPositionTargetSpecify=on  PzPositionTargetPriority=High  PzPositionTargetValue=waypoints(3,1)  PzPositionTargetValueUnits=m  PzVelocityTargetSpecify=off  PzVelocityTargetPriority=High  PzVelocityTargetValue=0  PzVelocityTargetValueUnits=m/s  PzEquilibriumPosition=0  PzEquilibriumPositionUnits=m  PzSpringStiffness=0  PzSpringStiffnessUnits=N/m  PzDampingCoefficient=0  PzDampingCoefficientUnits=N/(m/s)  PzLowerLimitSpecify=off  PzLowerLimitBound=-1  PzLowerLimitBoundUnits=m  PzLowerLimitStiffness=1e6  PzLowerLimitStiffnessUnits=N/m  PzLowerLimitDamping=1e3  PzLowerLimitDampingUnits=N/(m/s)  PzLowerLimitTransitionRegionWidth=1e-4  PzLowerLimitTransitionRegionWidthUnits=m  PzUpperLimitSpecify=off  PzUpperLimitBound=1  PzUpperLimitBoundUnits=m  PzUpperLimitStiffness=1e6  PzUpperLimitStiffnessUnits=N/m  PzUpperLimitDamping=1e3  PzUpperLimitDampingUnits=N/(m/s)  PzUpperLimitTransitionRegionWidth=1e-4  PzUpperLimitTransitionRegionWidthUnits=m  PzTorqueActuationMode=NoTorque  PzMotionActuationMode=ComputedMotion  PzSensePosition=on  PzSenseVelocity=on  PzSenseAcceleration=off  PzSenseTorqueForce=off  PzSenseLowerLimitTorqueForce=off  PzSenseUpperLimitTorqueForce=off
  Spherical Joint : sm_lib/Joints/Spherical Joint  JointMode=Normal  CompositeWrenchDir=FollowerOnBase  CompositeWrenchFrame=BaseFrame  SenseConstraintForce=off  SenseConstraintTorque=off  SenseTotalForce=off  SenseTotalTorque=off  PositionTargetSpecify=on  PositionTargetPriority=High  PositionTargetRotationMethod=RotationSequence  PositionTargetFollAlignAxisA=+X  PositionTargetBaseAlignAxisA=+Y  PositionTargetFollAlignAxisB=+Y  PositionTargetBaseAlignAxisB=+Z  PositionTargetRotationStandardAxis=+Z  PositionTargetRotationAngle=0.0  PositionTargetRotationAngleUnits=deg  PositionTargetRotationArbitraryAxis=[0 0 1]  PositionTargetRotationSequenceAxes=FollowerAxes  PositionTargetRotationSequence=XYX  PositionTargetRotationSequenceAngles=[0 0 0]  PositionTargetRotationSequenceAnglesUnits=deg  PositionTargetRotationMatrix=[1 0 0; 0 1 0; 0 0 1]  PositionTargetQuaternion=[1 0 0 0]  VelocityTargetSpecify=off  VelocityTargetPriority=High  VelocityTargetValue=[0 0 0]  VelocityTargetValueUnits=deg/s  VelocityTargetInFollowerFrame=on  EqPosRotationMethod=None  EqPosFollAlignAxisA=+X  EqPosBaseAlignAxisA=+Y  EqPosFollAlignAxisB=+Y  EqPosBaseAlignAxisB=+Z  EqPosRotationStandardAxis=+Z  EqPosRotationAngle=0.0  EqPosRotationAngleUnits=deg  EqPosRotationArbitraryAxis=[0 0 1]  EqPosRotationSequenceAxes=FollowerAxes  EqPosRotationSequence=XYX  EqPosRotationSequenceAngles=[0 0 0]  EqPosRotationSequenceAnglesUnits=deg  EqPosRotationMatrix=[1 0 0; 0 1 0; 0 0 1]  EqPosQuaternion=[1 0 0 0]  SpringStiffness=0  SpringStiffnessUnits=N*m/deg  DampingCoefficient=0  DampingCoefficientUnits=N*m/(deg/s)  LowerLimitSpecify=off  LowerLimitBound=15  LowerLimitBoundUnits=deg  LowerLimitStiffness=1e4  LowerLimitStiffnessUnits=N*m/deg  LowerLimitDamping=10  LowerLimitDampingUnits=N*m/(deg/s)  LowerLimitTransitionRegionWidth=0.1  LowerLimitTransitionRegionWidthUnits=deg  UpperLimitSpecify=off  UpperLimitBound=45  UpperLimitBoundUnits=deg  UpperLimitStiffness=1e4  UpperLimitStiffnessUnits=N*m/deg  UpperLimitDamping=10  UpperLimitDampingUnits=N*m/(deg/s)  UpperLimitTransitionRegionWidth=0.1  UpperLimitTransitionRegionWidthUnits=deg  TorqueActuationMode=NoTorque  ActuateTorqueX=off  ActuateTorqueY=off  ActuateTorqueZ=off  ActuateTorque=off  ActuationFrame=BaseFrame  SensePosition=off  SenseVelocityX=on  SenseVelocityY=on  SenseVelocityZ=on  SenseVelocity=off  SenseAccelerationX=off  SenseAccelerationY=off  SenseAccelerationZ=off  SenseAcceleration=off  SenseLowerLimitTorqueMag=off  SenseUpperLimitTorqueMag=off  SensingFrame=FollowerFrame
  C : PMIOPort  Side=Right
  F : PMIOPort  Port=2  Side=Right
  px : PMIOPort  Port=3  Side=Right
  vx : PMIOPort  Port=4  Side=Right
  B : PMIOPort  Port=5  Side=Left
  py : PMIOPort  Port=6  Side=Right
  vy : PMIOPort  Port=7  Side=Right
  pz : PMIOPort  Port=8  Side=Right
  vz : PMIOPort  Port=9  Side=Right
  nRoll : PMIOPort  Port=10  Side=Right
  nPitch : PMIOPort  Port=11  Side=Right
  nYaw : PMIOPort  Port=12  Side=Right
  connections:
  Cartesian Joint/LConn1 -- B/RConn1
  Cartesian Joint/RConn2 -- px/RConn1
  Cartesian Joint/RConn5 -- vy/RConn1
  Cartesian Joint/RConn1 -- C/RConn1 -- Spherical Joint/LConn1
  Cartesian Joint/RConn7 -- vz/RConn1
  Spherical Joint/RConn1 -- F/RConn1
  Cartesian Joint/RConn4 -- py/RConn1
  Cartesian Joint/RConn6 -- pz/RConn1
  Cartesian Joint/RConn3 -- vx/RConn1
  nYaw/RConn1 -- Spherical Joint/RConn4
  Spherical Joint/RConn2 -- nRoll/RConn1
  Spherical Joint/RConn3 -- nPitch/RConn1

== system t_drone/Quadcopter/6 DOF/R to X-Y-Z Extrinsic ==
  note: The sensor implemented here computes roll / pitch / yaw values assuming they correpsond to X, Y, and Z rotations, applied in that order and using  *extrinsic* rotations.  That is, the rotations are applied about the fixed (non-rotated) axes of the base frame.   There are many other possible conventions, but the computations of angles has the same basic structure for any of them.  The only differences would be which elements of the rotation matrix are picked off for analysis, and which signals are negated.
      |
      | This implementation does not handle the gimbal-lock case robustly, which occurs when the Y (pitch) rotation is +/-90 degrees.  Handling this case requires a more complex computation,
      | but it can be done with a few more trig blocks and selectors.
  R : Inport
  nYaw : Inport  Port=2
  Asin : Trigonometry  Operator=asin
  Atan1 : Trigonometry  Operator=atan2
  Atan2 : Trigonometry  Operator=atan2
  Demux : Demux  Outputs=2
  Demux1 : Demux  Outputs=2
  Multiply2 : Gain  Gain=-1
  Mux : Mux  Inputs=2
  "R(3, 1)" : Selector  NumberOfDimensions=2  InputPortWidth=3  IndexOptions=Index vector (dialog),Index vector (dialog)  Indices=3,1  OutputSizes=1,1
  "R(3, 2:3)" : Selector  NumberOfDimensions=2  InputPortWidth=3  IndexOptions=Index vector (dialog),Index vector (dialog)  Indices=3,[2 3]  OutputSizes=1,1
  "R([2 1], 1)" : Selector  NumberOfDimensions=2  InputPortWidth=3  IndexOptions=Index vector (dialog),Index vector (dialog)  Indices=[2 1],1  OutputSizes=1,1
  Reshape : Reshape
  Reshape1 : Reshape
  Reshape2 : Reshape  OutputDimensionality=Customize  OutputDimensions=1
  Scope : Scope  NumInputPorts=2
      settings: ActiveDisplayYMinimum=-4.33662  ActiveDisplayYMaximum=7.61477  DataLoggingVariableName=ScopeData2
  Unwrap : Subsystem
  yaw : Outport  VectorParamsAs1DForOutWhenUnconnected=off
  pitch : Outport  Port=2  VectorParamsAs1DForOutWhenUnconnected=off
  roll : Outport  Port=3  VectorParamsAs1DForOutWhenUnconnected=off
  yawWr : Outport  Port=4  VectorParamsAs1DForOutWhenUnconnected=off
  wires:
  Demux/1 -> Atan2/1
  Demux1/2 -> Atan1/2
  Demux/2 -> Atan2/2
  Atan2/1 -> Reshape2/1
  "R(3, 1)"/1 -> Multiply2/1
  Asin/1 -> Reshape1/1
  R/1 -> "R(3, 2:3)"/1, "R(3, 1)"/1, "R([2 1], 1)"/1
  Demux1/1 -> Atan1/1
  "R([2 1], 1)"/1 -> Demux1/1
  Multiply2/1 -> Asin/1
  "R(3, 2:3)"/1 -> Demux/1
  Atan1/1 -> Reshape/1
  Reshape1/1 -> pitch/1
  Reshape2/1 -> roll/1
  Reshape/1 -> Mux/1, yawWr/1, Unwrap/1(angle)
  Unwrap/1(unwrapped) -> Mux/2, yaw/1
  nYaw/1 -> Scope/2, Unwrap/2(w)
  Mux/1 -> Scope/1

== system t_drone/Quadcopter/6 DOF/Roll Pitch ==
  R : Inport
  Calculate aPitch : Subsystem
  Calculate aRoll : Subsystem
  "Flip sign for -x axis " : Gain  Gain=-1
  Select x axis : Selector  NumberOfDimensions=2  InputPortWidth=2  IndexOptions=Index vector (dialog),Index vector (dialog)  Indices=[1 2 3],1  OutputSizes=1,1
  Select y axis : Selector  NumberOfDimensions=2  InputPortWidth=2  IndexOptions=Index vector (dialog),Index vector (dialog)  Indices=[1 2 3],2  OutputSizes=1,1
  Transfer Fcn : TransferFcn  Numerator=[1 0]  Denominator=[0.01 1]
  Transfer Fcn1 : TransferFcn  Numerator=[1 0]  Denominator=[0.01 1]
  aRoll : Outport  VectorParamsAs1DForOutWhenUnconnected=off
  aPitch : Outport  Port=2  VectorParamsAs1DForOutWhenUnconnected=off
  nRoll : Outport  Port=3  VectorParamsAs1DForOutWhenUnconnected=off
  nPitch : Outport  Port=4  VectorParamsAs1DForOutWhenUnconnected=off
  wires:
  Calculate aPitch/1(Angle) -> "Flip sign for -x axis "/1
  Select x axis/1 -> Calculate aPitch/2(uvec)
  R/1 -> Select y axis/1, Select x axis/1
  Select y axis/1 -> Calculate aRoll/1(uvec)
  "Flip sign for -x axis "/1 -> aPitch/1, Transfer Fcn1/1
  Calculate aRoll/1(Angle) -> Transfer Fcn/1, aRoll/1, Calculate aPitch/1(Roll Angle)
  Transfer Fcn/1 -> nRoll/1
  Transfer Fcn1/1 -> nPitch/1

== system t_drone/Quadcopter/Body/Arm1 Contact Point ==
  Contact Force A2 : sm_lib/Forces and Torques/Spatial Contact Force  SenseSeparationDistance=off  NormalForceType=SmoothSpringDamper  NormalStiffness=pkgGrndStiff  NormalStiffnessUnits=N/m  NormalDamping=pkgGrndDamp  NormalDampingUnits=N/(m/s)  NormalTransitionRegionWidth=pkgGrndTransW  NormalTransitionRegionWidthUnits=m  FrictionType=SmoothStickSlip  CoefficientOfStaticFriction=0.5  CoefficientOfDynamicFriction=0.3  FrictionalCriticalVelocity=1e-2  FrictionalCriticalVelocityUnits=m/s  SenseContactSignal=off  SensePenetrationDepth=off  SenseNormalVelocity=off  SenseTangentialVelocity=off  SensingForceTorqueDirection=BaseOnFollower  SensingForceTorqueResolutionFrame=ContactFrame  SenseNormalForce=off  SenseNormalForceMagnitude=off  SenseNormalTorque=off  SenseFrictionalForce=off  SenseFrictionalForceMagnitude=off  SenseFrictionalTorque=off  SenseTotalForce=off  SenseTotalTorque=off  SenseContactBaseRotation=off  SenseContactBaseTranslation=off  SenseContactFollowerRotation=off  SenseContactFollowerTranslation=off  ZeroCrossDetectContactStartAndEnd=off
  Point A2 : sm_lib/Curves and Surfaces/Point  GraphicType=Marker  MarkerShape=Sphere  MarkerSize=10  GraphicVisPropType=SimpleVisualProperties  GraphicDiffuseColor=[0.5 0.5 0.5]  GraphicOpacity=0  GraphicSpecularColor=[0.5 0.5 0.5 1.0]  GraphicAmbientColor=[0.15 0.15 0.15 1.0]  GraphicEmissiveColor=[0.0 0.0 0.0 1.0]  GraphicShininess=75
  Rigid Transform5 : sm_lib/Frames and Transforms/Rigid Transform  RotationMethod=None  FollAlignAxisA=+X  BaseAlignAxisA=+Y  FollAlignAxisB=+Y  BaseAlignAxisB=+Z  RotationStandardAxis=+Z  RotationAngle=0  RotationAngleUnits=deg  RotationArbitraryAxis=[0 0 1]  RotationSequenceAxes=FollowerAxes  RotationSequence=XYX  RotationSequenceAngles=[0 0 0]  RotationSequenceAnglesUnits=deg  RotationMatrix=[1 0 0;0 1 0;0 0 1]  Quaternion=[1 0 0 0]  TranslationMethod=Cartesian  TranslationCartesianOffset=[0 40 40]  TranslationCartesianOffsetUnits=mm  TranslationStandardAxis=+Z  TranslationStandardOffset=0  TranslationStandardOffsetUnits=m  TranslationROffset=0  TranslationROffsetUnits=m  TranslationThetaOffset=0  TranslationThetaOffsetUnits=deg  TranslationZOffset=0  TranslationZOffsetUnits=m
  F : PMIOPort  Side=Right
  B : PMIOPort  Port=2  Side=Left
  connections:
  Point A2/LConn1 -- Rigid Transform5/RConn1
  Point A2/RConn1 -- Contact Force A2/LConn1
  Contact Force A2/RConn1 -- F/RConn1
  Rigid Transform5/LConn1 -- B/RConn1

== system t_drone/Quadcopter/Body/Arm2 Contact Point ==
  Contact Force A3 : sm_lib/Forces and Torques/Spatial Contact Force  SenseSeparationDistance=off  NormalForceType=SmoothSpringDamper  NormalStiffness=pkgGrndStiff  NormalStiffnessUnits=N/m  NormalDamping=pkgGrndDamp  NormalDampingUnits=N/(m/s)  NormalTransitionRegionWidth=pkgGrndTransW  NormalTransitionRegionWidthUnits=m  FrictionType=SmoothStickSlip  CoefficientOfStaticFriction=0.5  CoefficientOfDynamicFriction=0.3  FrictionalCriticalVelocity=1e-2  FrictionalCriticalVelocityUnits=m/s  SenseContactSignal=off  SensePenetrationDepth=off  SenseNormalVelocity=off  SenseTangentialVelocity=off  SensingForceTorqueDirection=BaseOnFollower  SensingForceTorqueResolutionFrame=ContactFrame  SenseNormalForce=off  SenseNormalForceMagnitude=off  SenseNormalTorque=off  SenseFrictionalForce=off  SenseFrictionalForceMagnitude=off  SenseFrictionalTorque=off  SenseTotalForce=off  SenseTotalTorque=off  SenseContactBaseRotation=off  SenseContactBaseTranslation=off  SenseContactFollowerRotation=off  SenseContactFollowerTranslation=off  ZeroCrossDetectContactStartAndEnd=off
  Point A3 : sm_lib/Curves and Surfaces/Point  GraphicType=Marker  MarkerShape=Sphere  MarkerSize=10  GraphicVisPropType=SimpleVisualProperties  GraphicDiffuseColor=[0.5 0.5 0.5]  GraphicOpacity=0  GraphicSpecularColor=[0.5 0.5 0.5 1.0]  GraphicAmbientColor=[0.15 0.15 0.15 1.0]  GraphicEmissiveColor=[0.0 0.0 0.0 1.0]  GraphicShininess=75
  Rigid Transform6 : sm_lib/Frames and Transforms/Rigid Transform  RotationMethod=None  FollAlignAxisA=+X  BaseAlignAxisA=+Y  FollAlignAxisB=+Y  BaseAlignAxisB=+Z  RotationStandardAxis=+Z  RotationAngle=0  RotationAngleUnits=deg  RotationArbitraryAxis=[0 0 1]  RotationSequenceAxes=FollowerAxes  RotationSequence=XYX  RotationSequenceAngles=[0 0 0]  RotationSequenceAnglesUnits=deg  RotationMatrix=[1 0 0;0 1 0;0 0 1]  Quaternion=[1 0 0 0]  TranslationMethod=Cartesian  TranslationCartesianOffset=[0 40 40]  TranslationCartesianOffsetUnits=mm  TranslationStandardAxis=+Z  TranslationStandardOffset=0  TranslationStandardOffsetUnits=m  TranslationROffset=0  TranslationROffsetUnits=m  TranslationThetaOffset=0  TranslationThetaOffsetUnits=deg  TranslationZOffset=0  TranslationZOffsetUnits=m
  F : PMIOPort  Side=Right
  B : PMIOPort  Port=2  Side=Left
  connections:
  Contact Force A3/RConn1 -- F/RConn1
  Point A3/RConn1 -- Contact Force A3/LConn1
  Point A3/LConn1 -- Rigid Transform6/RConn1
  Rigid Transform6/LConn1 -- B/RConn1

== system t_drone/Quadcopter/Body/Arm3 Contact Point ==
  Contact Force A1 : sm_lib/Forces and Torques/Spatial Contact Force  SenseSeparationDistance=off  NormalForceType=SmoothSpringDamper  NormalStiffness=pkgGrndStiff  NormalStiffnessUnits=N/m  NormalDamping=pkgGrndDamp  NormalDampingUnits=N/(m/s)  NormalTransitionRegionWidth=pkgGrndTransW  NormalTransitionRegionWidthUnits=m  FrictionType=SmoothStickSlip  CoefficientOfStaticFriction=0.5  CoefficientOfDynamicFriction=0.3  FrictionalCriticalVelocity=1e-2  FrictionalCriticalVelocityUnits=m/s  SenseContactSignal=off  SensePenetrationDepth=off  SenseNormalVelocity=off  SenseTangentialVelocity=off  SensingForceTorqueDirection=BaseOnFollower  SensingForceTorqueResolutionFrame=ContactFrame  SenseNormalForce=off  SenseNormalForceMagnitude=off  SenseNormalTorque=off  SenseFrictionalForce=off  SenseFrictionalForceMagnitude=off  SenseFrictionalTorque=off  SenseTotalForce=off  SenseTotalTorque=off  SenseContactBaseRotation=off  SenseContactBaseTranslation=off  SenseContactFollowerRotation=off  SenseContactFollowerTranslation=off  ZeroCrossDetectContactStartAndEnd=off
  Point A1 : sm_lib/Curves and Surfaces/Point  GraphicType=Marker  MarkerShape=Sphere  MarkerSize=10  GraphicVisPropType=SimpleVisualProperties  GraphicDiffuseColor=[0.5 0.5 0.5]  GraphicOpacity=0  GraphicSpecularColor=[0.5 0.5 0.5 1.0]  GraphicAmbientColor=[0.15 0.15 0.15 1.0]  GraphicEmissiveColor=[0.0 0.0 0.0 1.0]  GraphicShininess=75
  Rigid Transform4 : sm_lib/Frames and Transforms/Rigid Transform  RotationMethod=None  FollAlignAxisA=+X  BaseAlignAxisA=+Y  FollAlignAxisB=+Y  BaseAlignAxisB=+Z  RotationStandardAxis=+Z  RotationAngle=0  RotationAngleUnits=deg  RotationArbitraryAxis=[0 0 1]  RotationSequenceAxes=FollowerAxes  RotationSequence=XYX  RotationSequenceAngles=[0 0 0]  RotationSequenceAnglesUnits=deg  RotationMatrix=[1 0 0;0 1 0;0 0 1]  Quaternion=[1 0 0 0]  TranslationMethod=Cartesian  TranslationCartesianOffset=[0 40 40]  TranslationCartesianOffsetUnits=mm  TranslationStandardAxis=+Z  TranslationStandardOffset=0  TranslationStandardOffsetUnits=m  TranslationROffset=0  TranslationROffsetUnits=m  TranslationThetaOffset=0  TranslationThetaOffsetUnits=deg  TranslationZOffset=0  TranslationZOffsetUnits=m
  F : PMIOPort  Side=Right
  B : PMIOPort  Port=2  Side=Left
  connections:
  Point A1/LConn1 -- Rigid Transform4/RConn1
  F/RConn1 -- Contact Force A1/RConn1
  Point A1/RConn1 -- Contact Force A1/LConn1
  Rigid Transform4/LConn1 -- B/RConn1
